simulink model "all_f16_0001_0001"  (R2026a)
settings: Solver=FixedStepDiscrete  FixedStep=0.01
settings Model: Creator=harry_31916  LastModifiedBy=harry_31916

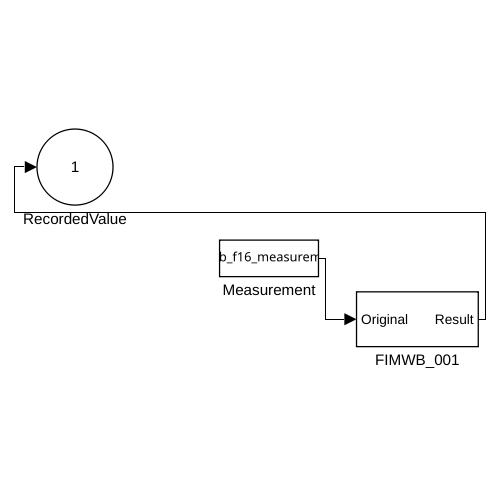
[thumbnail: Simulink's stored preview of the top-level diagram]
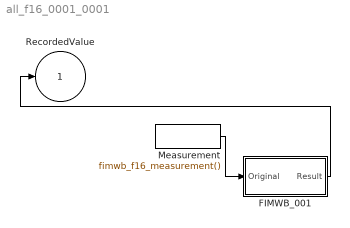
== system all_f16_0001_0001 ==
  FIMWB_001 : Subsystem  Tag=fimwb.fault.1
  Measurement : FromWorkspace  VariableName=fimwb_f16_measurement()  SampleTime=0.01  OutputAfterFinalValue=Holding final value
  RecordedValue : Outport
  wires:
  Measurement/1 -> FIMWB_001/1(Original)
  FIMWB_001/1(Result) -> RecordedValue/1

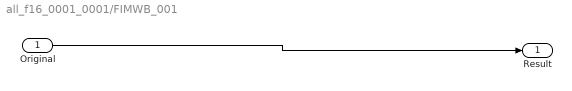
== system all_f16_0001_0001/FIMWB_001 ==
  Original : Inport
  Result : Outport
  wires:
  Original/1 -> Result/1
